simulink model "Dual_Clutch_Trans_SDO"  (R2025a)
settings: Solver=ode1  StartTime=0.0  StopTime=15  MaxStep=0.1  RelTol=1e-3  EnableMultiTasking=on
PreLoadFcn:
  | load UrbanCycle1;
  | load UrbanCycle2;
  | load UrbanCycle3;
  | load UrbanCycle4;
  | load UrbanCycle5;
  | load UrbanCycle6;
  | load UrbanCycle7;
  | load UrbanCycle8;
  | Shift_Gear_Delay = 50;
  | Ratio_Time_Const = 0.1;
  | Drive_Cycle_Num = 7;
  | load RefRPMData;
PostLoadFcn:
  | warning off Simulink:SampleTime:TsPropEnabOutputsChangeNotAligned;
  | warning off Simulink:blocks:MatchingFromNotFound
  | warning off Simulink:blocks:MatchingGotoNotFound
  | warning off Simulink:Engine:OutputNotConnected
  | warning off Simulink:Engine:LineWithoutDst
  | warning off Simulink:Engine:UINotUpdatedDuringRapidAccelSim
  | warning off Simulink:Commands:SetParamLinkChangeWarn
  | warning off Simulink:Engine:SaveWithParameterizedLinks_Warning
undefined symbols (not defined in the file or in its folder): DCT_Param, Downshift_Speeds, sigbuilder_block, Upshift_Speeds
libraries: fl_lib x5, nesl_utility x4, sdl_lib x2, simulink x2, DCT_Vehicle_Dynamics_Lib x2, Engine_Lib x1, slpidlib x1
(part 1 of 2)
Description:
  | Vehicle With Dual Clutch Transmission
  | 
  | The vehicle simulated in this demo has a five-speed automatic dual-clutch
  | transmission. The transmission controller converts the pedal deflection
  | into a demanded torque. This demanded torque is then passed to the
  | engine management. The pedal deflection and the vehicle speed are also
  | used by the transmission controller to determine when the gear shifts
  | should occur. Gear shifts are implemented via the two clutches, one clutch
  | pressure being ramped up as the other clutch pressure is ramped down.
  | Gear pre-selection is used to ensure that the correct gear is fully selected
  | before the on-going clutch is enabled. Double-click on the two blocks
  | labeled "Configure for ...." to switch between variable and fixed-step solvers.
  | 
  | 
  | Copyright 2008-2025 The MathWorks, Inc.
settings Model: ParamWorkspaceSource=ReferencedWorkspace  ExtModeTrigDuration=200  ExtModeLogAll=off  TunableVars=Downshift_Speeds,Pedal_Positions,Upshift_Speeds  TunableVarsStorageClass=Auto,Auto,Auto  TunableVarsTypeQualifier=,,  Creator=MathWorks  LastModifiedBy=smiller
settings SolverCC: MaxConsecutiveZCs=10  MaxConsecutiveMinStep=5  AlgebraicLoopSolver=TrustRegion  AutoInsertRateTranBlk=on
settings DataIOCC: LimitDataPoints=on  MaxDataPoints=1  SaveFormat=StructureWithTime  SaveOutput=off  DSMLogging=off  SaveTime=off  ReturnWorkspaceOutputs=off  SignalLoggingName=SDO_logsout
settings OptimizationCC: BlockReduction=off  OptimizeBlockIOStorage=off  BufferReuse=off  ReuseModelBlockBuffer=off  GlobalBufferReuse=off  ExpressionFolding=off  ExpressionDepthLimit=2147483647.0  LocalBlockOutputs=off  OptimizeDataStoreBuffers=off  BusAssignmentInplaceUpdate=off
settings DebuggingCC: AlgebraicLoopMsg=error  UnderspecifiedInitializationDetection=Classic  MergeDetectMultiDrivingBlocksExec=none  IgnoredZcDiagnostic=none  MultiTaskRateTransMsg=warning  FcnCallInpInsideContextMsg=warning  UnconnectedInputMsg=warning  UnconnectedOutputMsg=warning  UnconnectedLineMsg=warning  AllowSymbolicDim=off  StateNameClashWarn=warning  PregeneratedLibrarySubsystemCodeDiagnostic=none  SFUnexpectedBacktrackingDiag=warning  SFNoUnconditionalDefaultTransitionDiag=warning  SFExecutionAtInitializationDiag=none  ArithmeticOperatorsInVariantConditions=warning
settings ModelReferenceCC: EnableRefExpFcnMdlSchedulingChecks=on  PropagateSignalLabelsOutOfModel=off
settings SFSimCC: SimUseLocalCustomCode=off  CustomCodeUndefinedFunction=UseInterfaceOnly
settings RTWCC: RTWUseLocalCustomCode=off  RTWCompilerOptimization=on  GPUComputeCapability=3.5  DLArmComputeVersion=19.05
settings CodeAppCC: StateflowObjectComments=on
settings GRTTargetCC: TargetLangStandard=C89/C90 (ANSI)
settings ConfigComp: CovMetricSettings=dw  CovSaveCumulativeToWorkspaceVar=on  CovSaveSingleToWorkspaceVar=on  CovExternalEMLEnable=off  CovSFcnEnable=off
settings SimscapeCC: ExplicitSolverDiagnosticOptions=none  SimscapeNormalizeSystem=off  SimscapeNominalValues="[{\"value\":\"10\",\"unit\":\"V\"},{\"value\":\"1\",\"unit\":\"A\"},{\"value\":\"10\",\"unit\":\"N*m\"},{\"value\":\"10\",\"unit\":\"bar\"},{\"value\":\"100\",\"unit\":\"kJ/kg\"},{\"value\":\"1\",\"unit\":\"kW\"},{\"value\":\"300\",\"unit\":\"K\"},{\"value\":\"100\",\"unit\":\"cm^3/s\"},{\"value\":\"1\",\"unit\":\"kN\"},{\"value\":\"1\",\"unit\":\"g/cm^3\"},{\"value\":\"1\",\"unit\":\"l\"},{\"value\":\"1\",\"unit\":\"cm^2\"},{\"value\":\"60\",\"unit\":\"Hz\"}]"  SimscapeLogLimitData=off  SimscapeLogDataHistory=50000.0

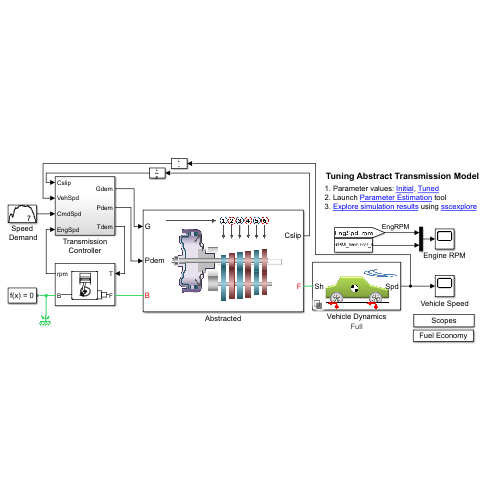
[thumbnail: Simulink's stored preview of the top-level diagram]
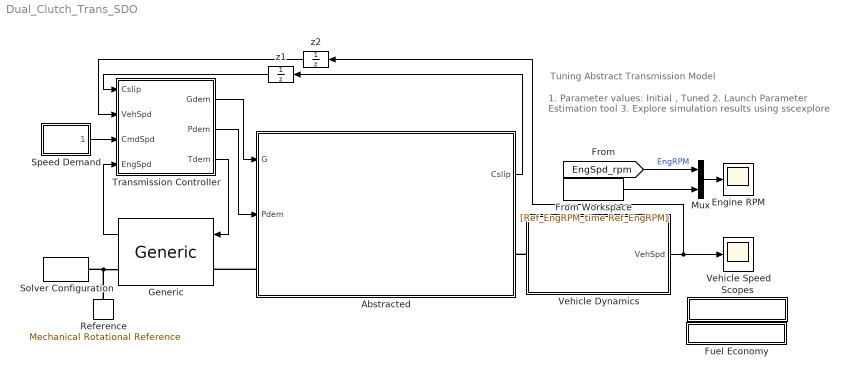
== system Dual_Clutch_Trans_SDO ==
  note: 1. Parameter values: Initial , Tuned
      | 2. Launch Parameter Estimation tool
      | 3. Explore simulation results using sscexplore
  note: Tuning Abstract Transmission Model
  Abstracted : Subsystem
      mask Display:
      | image(imread('DCT_Transmission_Abstracted_IMAGE2.jpg'));
      | port_label('input',1,'G')
      | port_label('input',2,'Pdem')
      | port_label('output',1,'Cslip')
      | color('red');
      | port_label('LConn',1,'B')
      | port_label('RConn',1,'F')
  Engine RPM : Scope
      settings: ActiveDisplayYMinimum=0  ActiveDisplayYMaximum=3000  DataLoggingMaxPoints=50000  DataLoggingVariableName=EngineRPM
  From Workspace : FromWorkspace  VariableName=[Ref_EngRPM_time Ref_EngRPM]  SampleTime=0.01
  Fuel Economy : Subsystem  mask(Data Acquisition){}
      mask Display: disp('Fuel Economy');
  Generic : Engine_Lib/Generic  SystemSampleTime=-1  VariantActivationTime=update diagram  EmptyChoice=off  PassThrough=off  PassThroughVariantControl=(default)  EmptyChoiceVariantControl=(default)  AllowFlexibleInterface=on  Latency=0  AutoFrameSizeCalculation=off
  Mux : Mux  Inputs=2
  Reference : fl_lib/Mechanical/Rotational Elements/Mechanical Rotational Reference
  Scopes : Subsystem
      mask Display: disp('Scopes')
  Solver Configuration : nesl_utility/Solver Configuration  PhysicalDomain=network_engine_domain  SubClassName=solver  LeftPortType=input  RightPortType=generic  Tones=[]  Harmonics=[]  SimulateNoise=off  Profile=off  UseLocalSampling=off  EnableSwitchedLinearOptims=on  FrequencyDomain=off  UseCCode=off  RelTol=0.001  AbsTol=1e-06  MinStep=1e-09  ToWorkspace=off  RevertToSquareIcSolve=off  NumHomotopyIterations=100  PhasorMode=off  PhasorModeNumHarmonics=1  ConsistencySolver=NEWTON_FTOL  IndexReductionMethod=DerivativeReplacement  DoDC=off  ResidualTolerance=1e-9  ConsistencyTolSource=GLOBAL  ConsistencyAbsTol=0.001  ConsistencyRelTol=0.001  ConsistencyTolFactor=0.001  UseLocalSolver=on  LocalSolverChoice=NE_BACKWARD_EULER_ADVANCER  ResolveIndetEquations=on  FunctionEvalNumThread=1  LocalSolverSampleTime=.005  DoFixedCost=on  MaxNonlinIter=2  MaxModeIter=2  ComputeImpulses=off  ImpulseIterations=2  LinearAlgebra=Sparse  LinearAlgebraNumThread=0  EquationFormulation=NE_TIME_EF  DelaysMemoryBudget=1024  AutomaticFiltering=on  FilteringTimeConstant=0.001  PartitionStorageMethod=AS_NEEDED  PartitionMemoryBudget=1024  PartitionMethod=FAST  MultibodyUseLocalSolver=off  MultibodyLocalSolverChoice=ODE1  MultibodyLocalSolverSampleTime=0.001
  Speed Demand : Subsystem
      mask Display:
      | plotstr=['UrbanCycle' evalin('base','num2str(Drive_Cycle_Num)')];
      | plot(evalin('base',[plotstr '.time']),evalin('base',[plotstr '.SpdKph']));
      | text(evalin('base',['0.7*max(' plotstr '.time)']),evalin('base',['0.25*max(' plotstr '.SpdKph)']),evalin('base','num2str(Drive_Cycle_Num)'));
  Transmission Controller : Subsystem
  Vehicle Dynamics : Subsystem  Variant=on  VariantControlMode=label  LabelModeActiveChoice=Full
      settings: AttributesFormatString=%<ActiveVariant>
      mask Display:
      | blk = Dual_Clutch_activeVariantBlock(gcb);
      | eval(get_param(blk, 'MaskDisplay'));
  Vehicle Speed : Scope
      settings: ActiveDisplayYMaximum=100  DataLoggingMaxPoints=50000  DataLoggingVariableName=VehSpd
  z1 : UnitDelay  SampleTime=0.01  HasFrameUpgradeWarning=on
  z2 : UnitDelay  SampleTime=0.01  HasFrameUpgradeWarning=on
  wires:
  Transmission Controller/2(Pdem) -> Abstracted/2(Pdem)
  Transmission Controller/1(Gdem) -> Abstracted/1(G)
  z1/1 -> Transmission Controller/1(Cslip)
  Generic/1 -> Transmission Controller/4(EngSpd)
  Abstracted/1(Cslip) -> z1/1
  Vehicle Dynamics/1(VehSpd) -> Vehicle Speed/1, z2/1
  Speed Demand/1(Speed Command) -> Transmission Controller/3(CmdSpd)
  z2/1 -> Transmission Controller/2(VehSpd)
  [EngSpd_rpm] -> Mux/1  "EngRPM"
  From Workspace/1 -> Mux/2
  Mux/1 -> Engine RPM/1
  Transmission Controller/3(Tdem) -> Generic/1
  connections:
  Generic/RConn1 -- Reference/LConn1 -- Solver Configuration/RConn1
  Abstracted/LConn1 -- Generic/LConn1
  Vehicle Dynamics/LConn1 -- Abstracted/RConn1

== system Dual_Clutch_Trans_SDO/Abstracted ==
  G : Inport
  Pdem : Inport  Port=2
  Clutches : Subsystem
      mask Display: image(imread('DCT_Clutches_Abstracted_IMAGE.jpg'));
  Gears : Subsystem
      mask Display: image(imread('DCT_Gears_Abstracted_IMAGE.jpg'));
  Shaft Inertia Output Shaft : fl_lib/Mechanical/Rotational Elements/Inertia  inertia=DCT_Param.Transmission.Shaft_Inertia_Output kg*m^2  num_ports=foundation.enum.numPorts2.one  w_specify=on  w_priority=High  w=DCT_Param.Transmission.Shaft_Velocity_Output rad/s  w_nominal_specify=off  w_nominal_value=1  w_nominal_unit=rad/s  t_specify=off  t_priority=High  t=0 N*m  t_nominal_specify=off  t_nominal_value=1  t_nominal_unit=N*m
  B : PMIOPort  Side=Left
  F : PMIOPort  Port=2  Side=Right
  Cslip : Outport  VectorParamsAs1DForOutWhenUnconnected=off
  wires:
  Pdem/1 -> Clutches/1(Pdem)
  Clutches/1(Cslip) -> Cslip/1
  G/1 -> Gears/1(G)
  connections:
  B/RConn1 -- Clutches/LConn1
  Clutches/RConn1 -- Gears/LConn1
  Gears/RConn1 -- F/RConn1 -- Shaft Inertia Output Shaft/LConn1

== system Dual_Clutch_Trans_SDO/Fuel Economy ==
  note: Fuel Economy
  (L/100 km) : Display
      settings: Decimation=decimation
  (MPG) : Display
      settings: Decimation=decimation
  (km/L) : Display
      settings: Decimation=decimation
  Calculate Fuel Economy : Subsystem
  Fuel Flow : Scope
      settings: ActiveDisplayYMinimum=0  ActiveDisplayYMaximum=7000  DataLoggingMaxPoints=50000  DataLoggingVariableName=Fuel_Flow_DATA
  Total Fuel Used (L) : Display
      settings: Decimation=decimation
  wires:
  [Fuel_Flow_gps] -> Fuel Flow/1, Calculate Fuel Economy/2(Fuel Flow g/s)
  Calculate Fuel Economy/2(Km/Liter) -> (km/L)/1
  Calculate Fuel Economy/4(Fuel Used (L)) -> Total Fuel Used (L)/1
  [VehSpd] -> Calculate Fuel Economy/1(Kph)
  Calculate Fuel Economy/3(MPG) -> (MPG)/1
  Calculate Fuel Economy/1(Liter/100Km) -> (L/100 km)/1

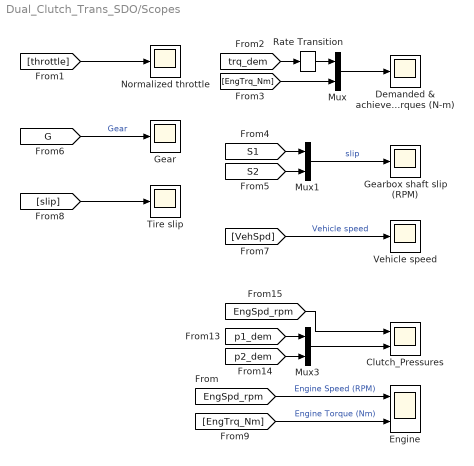
== system Dual_Clutch_Trans_SDO/Scopes ==
  Clutch_Pressures : Scope  NumInputPorts=2
      settings: ActiveDisplayYMinimum=0  ActiveDisplayYMaximum=6000  DataLoggingMaxPoints=50000  DataLoggingVariableName=Torque1
  Demanded & achieved torques (N-m) : Scope
      settings: TimeSpan=30  ActiveDisplayYMinimum=0  ActiveDisplayYMaximum=200  DataLoggingMaxPoints=50000  DataLoggingVariableName=Torque  DataLoggingSaveFormat=Array
  Engine : Scope  NumInputPorts=2
      settings: ActiveDisplayYMinimum=0  ActiveDisplayYMaximum=6000  DataLoggingMaxPoints=50000  DataLoggingVariableName=Engine_DATA
  Gear : Scope
      settings: ActiveDisplayYMinimum=0  ActiveDisplayYMaximum=5.5  DataLoggingMaxPoints=50000  DataLoggingVariableName=CurrentGear_DATA
  Gearbox shaft slip (RPM) : Scope
      settings: ActiveDisplayYMinimum=-4000  ActiveDisplayYMaximum=4000  DataLoggingMaxPoints=50000
  Mux : Mux  Inputs=2
  Mux1 : Mux  Inputs=2
  Mux3 : Mux  Inputs=2
  Normalized throttle : Scope
      settings: TimeSpan=30  ActiveDisplayYMinimum=0  ActiveDisplayYMaximum=1  DataLoggingMaxPoints=50000
  Rate Transition : RateTransition
  Tire slip : Scope
      settings: ActiveDisplayYMinimum=0  ActiveDisplayYMaximum=0.04  DataLoggingMaxPoints=500000  DataLoggingVariableName=TireSlip  DataLoggingSaveFormat=Array
  Vehicle speed : Scope
      settings: ActiveDisplayYMaximum=50  DataLoggingMaxPoints=50000  DataLoggingVariableName=VehicleSpeed_DATA
  wires:
  [throttle] -> Normalized throttle/1
  Mux/1 -> Demanded & achieved torques (N-m)/1
  [EngTrq_Nm] -> Mux/2
  Mux1/1 -> Gearbox shaft slip (RPM)/1  "slip"
  [S1] -> Mux1/1
  [S2] -> Mux1/2
  [G] -> Gear/1  "Gear"
  [VehSpd] -> Vehicle speed/1  "Vehicle speed"
  [slip] -> Tire slip/1
  Mux3/1 -> Clutch_Pressures/2
  [p1_dem] -> Mux3/1
  [p2_dem] -> Mux3/2
  [EngSpd_rpm] -> Clutch_Pressures/1
  [trq_dem] -> Rate Transition/1
  Rate Transition/1 -> Mux/1
  [EngSpd_rpm] -> Engine/1  "Engine Speed (RPM)"
  [EngTrq_Nm] -> Engine/2  "Engine Torque (Nm)"

== system Dual_Clutch_Trans_SDO/Speed Demand ==
  "10-15 mode " : Subsystem  Tag=STV Subsys  LoadFcn=sigbuilder_block('load');  StartFcn=sigbuilder_block('start');  StopFcn=sigbuilder_block('stop');  ClipboardFcn=sigbuilder_block('clipboard');  mask(Sigbuilder block){tuvar=[0:10]}
      mask help: Sigbuilder GUI
      mask init:
      | if ~strcmp(get_param(bdroot(gcbh),'SimulationStatus'),'stopped') tuvar = sigbuilder_block('maskInit'); end
      settings: CopyFcn=sigbuilder_block('copy');  DeleteFcn=sigbuilder_block('delete');  ModelCloseFcn=sigbuilder_block('modelClose');  PreSaveFcn=sigbuilder_block('preSave');  PauseFcn=sigbuilder_block('pause')  ContinueFcn=sigbuilder_block('continue')  NameChangeFcn=sigbuilder_block('namechange');  OpenFcn=sigbuilder_block('open',[561.75 178.5 550.5 399 ]);  CloseFcn=sigbuilder_block('close');
      mask Display: plot(0, 0, 100, 100,[2, 2, 32, 32, 2], [68, 8, 8, 68, 68],[32, 2], [38, 38], [32, 19, 2],[53, 60, 44], [32, 17, 17, 2],[16, 16, 31, 31]);txt = getActiveGroup(gcbh);text(2, 100, txt,'verticalAlignment', 'top');
  FTP75 : FromWorkspace  VariableName=[UrbanCycle4.time UrbanCycle4.SpdKph]
  FTP75 Transient : FromWorkspace  VariableName=[UrbanCycle8.time UrbanCycle8.SpdKph]
  FTP75 short : FromWorkspace  VariableName=[UrbanCycle7.time UrbanCycle7.SpdKph]
  Multiport Switch : MultiPortSwitch  Inputs=8  SaturateOnIntegerOverflow=off  InputSameDT=off
  Select Cycle : Constant  Value=Drive_Cycle_Num
  Urban Cycle 1 : FromWorkspace  VariableName=[UrbanCycle1.time UrbanCycle1.SpdKph]
  Urban Cycle 2 : FromWorkspace  VariableName=[UrbanCycle2.time UrbanCycle2.SpdKph]
  Urban Cycle 3 : FromWorkspace  VariableName=[UrbanCycle3.time UrbanCycle3.SpdKph]
  Wide Open Throttle : FromWorkspace  VariableName=[UrbanCycle4.time UrbanCycle4.SpdKph]
  Speed Command : Outport  VectorParamsAs1DForOutWhenUnconnected=off
  wires:
  Urban Cycle 3/1 -> Multiport Switch/4
  Select Cycle/1 -> Multiport Switch/1
  Urban Cycle 2/1 -> Multiport Switch/3
  Urban Cycle 1/1 -> Multiport Switch/2
  FTP75/1 -> Multiport Switch/5
  "10-15 mode "/1(Target speed) -> Multiport Switch/6
  Multiport Switch/1 -> Speed Command/1
  FTP75 short/1 -> Multiport Switch/8
  Wide Open Throttle/1 -> Multiport Switch/7
  FTP75 Transient/1 -> Multiport Switch/9

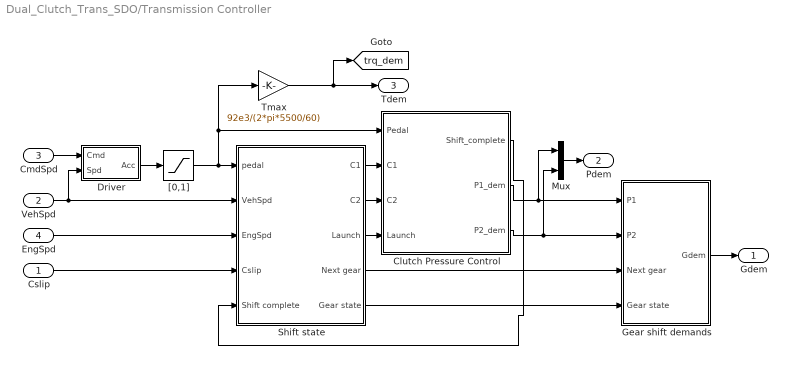
== system Dual_Clutch_Trans_SDO/Transmission Controller ==
  Cslip : Inport
  VehSpd : Inport  Port=2
  CmdSpd : Inport  Port=3
  EngSpd : Inport  Port=4
  Clutch Pressure Control : Subsystem
  Driver : Subsystem
  Gear shift demands : Subsystem
  Mux : Mux  Inputs=2
  Shift state : Subsystem
  Tmax : Gain  Gain=92e3/(2*pi*5500/60)  SaturateOnIntegerOverflow=on  OutDataTypeStr=Inherit: Same as input  ParamDataTypeStr=Inherit: Same as input
  "[0,1]" : Saturate  UpperLimit=1  LowerLimit=0
  Gdem : Outport  VectorParamsAs1DForOutWhenUnconnected=off
  Pdem : Outport  Port=2  VectorParamsAs1DForOutWhenUnconnected=off
  Tdem : Outport  Port=3  VectorParamsAs1DForOutWhenUnconnected=off
  tag scope: trq_dem=global
  wires:
  "[0,1]"/1 -> Shift state/1(pedal), Clutch Pressure Control/1(Pedal), Tmax/1
  VehSpd/1 -> Shift state/2(VehSpd), Driver/2(Spd)
  EngSpd/1 -> Shift state/3(EngSpd)
  Cslip/1 -> Shift state/4(Cslip)
  Shift state/5(Gear state) -> Gear shift demands/4(Gear state)
  Shift state/4(Next gear) -> Gear shift demands/3(Next gear)
  Gear shift demands/1(Gdem) -> Gdem/1
  Shift state/1(C1) -> Clutch Pressure Control/2(C1)
  Shift state/2(C2) -> Clutch Pressure Control/3(C2)
  Shift state/3(Launch) -> Clutch Pressure Control/4(Launch)
  Clutch Pressure Control/1(Shift_complete) -> Shift state/5(Shift complete)
  Clutch Pressure Control/3(P2_dem) -> Gear shift demands/2(P2), Mux/2
  Clutch Pressure Control/2(P1_dem) -> Gear shift demands/1(P1), Mux/1
  Tmax/1 -> Tdem/1, [trq_dem]
  Mux/1 -> Pdem/1
  CmdSpd/1 -> Driver/1(Cmd)
  Driver/1(Acc) -> "[0,1]"/1

== system Dual_Clutch_Trans_SDO/Vehicle Dynamics ==
  note: Variant Subsystems
  Full : DCT_Vehicle_Dynamics_Lib/Full  SystemSampleTime=-1  VariantControl=Full  VariantActivationTime=update diagram  EmptyChoice=off  PassThrough=off  PassThroughVariantControl=(default)  EmptyChoiceVariantControl=(default)  AllowFlexibleInterface=on  Latency=0  AutoFrameSizeCalculation=off
  Simple : DCT_Vehicle_Dynamics_Lib/Simple  VariantControl=Simple  mass=DCT_Param.Vehicle.Mass  area=DCT_Param.Vehicle.Frontal_Area  Cd=DCT_Param.Vehicle.Aero_Drag_Coeff  radius=DCT_Param.Vehicle.Tire.Radius  wheel_inertia=DCT_Param.Vehicle.Tire.Inertia  gear_ratio=DCT_Param.Vehicle.Final_Drive_Ratio
  Drive Shaft : PMIOPort  Side=Left
  VehSpd : Outport  VectorParamsAs1DForOutWhenUnconnected=off

== system Dual_Clutch_Trans_SDO/Abstracted/Clutches ==
  Pdem : Inport
  Clutch Odd Gears : sdl_lib/Clutches/Disc Friction Clutch  geometry_model=1  r_eff=DCT_Param.Clutch.Torque_Radius mm  d_o=150 mm  d_i=100 mm  nS=DCT_Param.Clutch.Num_Friction_Surfaces  piston_area=DCT_Param.Clutch.Engagement_Piston_Area m^2  unidirectional=0  friction_model=1  mu_w_vector=[ 0 0.1 0.2 0.3 0.4 0.5 1 2 5 10 100 1000 ] rad/s  temperature_TLU=[280.0, 300.0, 320.0] K  mu_static=DCT_Param.Clutch.Static_Friction_Coeff  mu_static_vector=[0.4, 0.38, 0.36]  mu_coulomb=DCT_Param.Clutch.Kinetic_Friction_Coeff  mu_coulomb_vector=[ 0.29 0.28 0.26 0.22 0.21 0.2 0.2 0.19 0.19 0.19 0.19 0.19 ]  mu_coulomb_temp_vector=[0.3, 0.28, 0.25]  mu_coulomb_matrix=[0.34, 0.32, 0.3; 0.3, 0.28, 0.25; 0.25, 0.2, 0.15]  mu_interp_method=1  mu_extrap_method=1  d_f=DCT_Param.Clutch.Derating_Factor  w_tol=DCT_Param.Clutch.Clutch_Velocity_Tolerance rad/s  pressure_min=DCT_Param.Clutch.Threshold_Pressure Pa  mu_visc=DCT_Param.Clutch.Drag_Torque_Coeff N*m/(rad/s)  initial_state_locked=0  thermal_mass=25 kJ/K  T_init=300 K
      settings: InternalSimscapePortConfiguration="{\"Bottom\":[],\"Left\":[{\"id\":\"P\",\"label\":\"P\",\"type\":\"input\"},{\"id\":\"B\",\"label\":\"B\",\"type\":\"foundation.mechanical.rotational.rotational\"}],\"Right\":[{\"id\":\"F\",\"label\":\"F\",\"type\":\"foundation.mechanical.rotational.rotational\"}],\"Top\":[]}"
  MinMax : MinMax  Function=max
  Mux : Mux  Inputs=2
  Odd Clutch Actuator : Subsystem
  Shaft Inertia All Gears : fl_lib/Mechanical/Rotational Elements/Inertia  inertia=DCT_Param.Transmission.Shaft_Inertia_Odd kg*m^2  num_ports=foundation.enum.numPorts2.one  w_specify=on  w_priority=High  w=DCT_Param.Transmission.Shaft_Velocity_Odd rad/s  w_nominal_specify=off  w_nominal_value=1  w_nominal_unit=rad/s  t_specify=off  t_priority=High  t=0 N*m  t_nominal_specify=off  t_nominal_value=1  t_nominal_unit=N*m
  Slip Sensor 2 : Constant  Value=0
  Slip sensor 1 : Subsystem
  Shaft : PMIOPort  Side=Right
  E : PMIOPort  Port=2  Side=Left
  Cslip : Outport  VectorParamsAs1DForOutWhenUnconnected=off
  wires:
  Slip sensor 1/1(S1) -> Mux/1
  Mux/1 -> Cslip/1
  Pdem/1 -> MinMax/1
  MinMax/1 -> Odd Clutch Actuator/1(Pdem)
  Slip Sensor 2/1 -> Mux/2
  connections:
  E/RConn1 -- Slip sensor 1/LConn1 -- Clutch Odd Gears/LConn2
  Odd Clutch Actuator/RConn1 -- Clutch Odd Gears/LConn1
  Slip sensor 1/RConn1 -- Clutch Odd Gears/RConn1 -- Shaft/RConn1 -- Shaft Inertia All Gears/LConn1

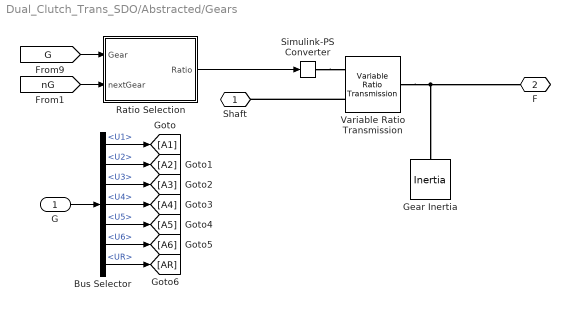
== system Dual_Clutch_Trans_SDO/Abstracted/Gears ==
  G : Inport
  Bus Selector : BusSelector  OutputSignals=U1,U2,U3,U4,U5,U6,UR
  Gear Inertia : fl_lib/Mechanical/Rotational Elements/Inertia  inertia=DCT_Param.Transmission.Gear_Inertia kg*m^2  num_ports=foundation.enum.numPorts2.one  w_specify=on  w_priority=High  w=0 rad/s  w_nominal_specify=off  w_nominal_value=1  w_nominal_unit=rad/s  t_specify=off  t_priority=High  t=0 N*m  t_nominal_specify=off  t_nominal_value=1  t_nominal_unit=N*m
  Ratio Selection : Subsystem
  Simulink-PS Converter : nesl_utility/Simulink-PS Converter  PhysicalDomain=network_engine_domain  SubClassName=ps_input  LeftPortType=input  RightPortType=output  PseudoPeriodic=off  Frequencies=[]  NoiseDistribution=none  NoiseParameters=[]  Unit=1  AffineConversion=off  FilteringAndDerivatives=zero  SimscapeFilterOrder=1  InputFilterTimeConstant=0.005  UdotUserProvided=0
  Variable Ratio Transmission : sdl_lib/Couplings & Drives/Variable Ratio Transmission  rotation_direction=3-2*(2)  kp=DCT_Param.Transmission.Abstract.Compliance N*m/rad  kv=DCT_Param.Transmission.Abstract.Damping N*m/(rad/s)  initial_torque=0 N*m  ratio_thr=0.01  losses_model=(1)-1  efficiency=0.85  pwr_thr=0.001 W  mu_visc=[ 0 0 ] N*m/(rad/s)
      settings: InternalSimscapePortConfiguration="{\"Bottom\":[],\"Left\":[{\"id\":\"ratio\",\"label\":\"r\",\"type\":\"input\"},{\"id\":\"B\",\"label\":\"B\",\"type\":\"foundation.mechanical.rotational.rotational\"}],\"Right\":[{\"id\":\"F\",\"label\":\"F\",\"type\":\"foundation.mechanical.rotational.rotational\"}],\"Top\":[]}"
  Shaft : PMIOPort  Side=Left
  F : PMIOPort  Port=2  Side=Right
  wires:
  [nG] -> Ratio Selection/2(nextGear)
  G/1 -> Bus Selector/1
  Bus Selector/1 -> [A1]  "<U1>"
  Bus Selector/2 -> [A2]  "<U2>"
  Bus Selector/3 -> [A3]  "<U3>"
  Bus Selector/4 -> [A4]  "<U4>"
  Bus Selector/5 -> [A5]  "<U5>"
  Bus Selector/6 -> [A6]  "<U6>"
  Bus Selector/7 -> [AR]  "<UR>"
  Ratio Selection/1(Ratio) -> Simulink-PS Converter/1
  [G] -> Ratio Selection/1(Gear)
  connections:
  Variable Ratio Transmission/LConn2 -- Shaft/RConn1
  Variable Ratio Transmission/RConn1 -- Gear Inertia/LConn1 -- F/RConn1
  Simulink-PS Converter/RConn1 -- Variable Ratio Transmission/LConn1

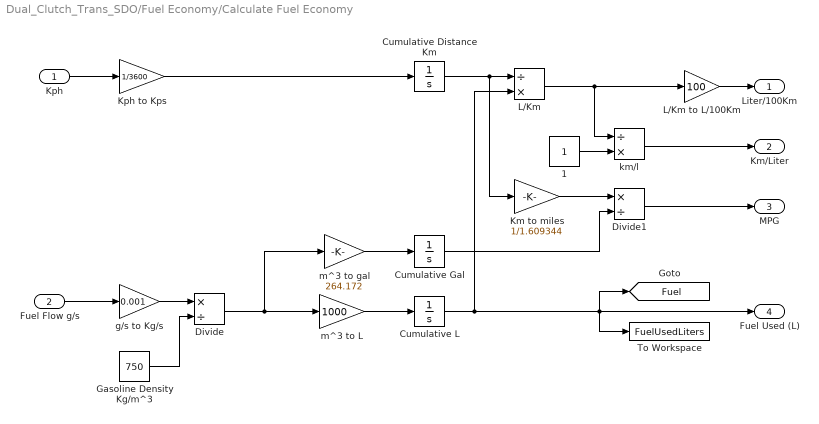
== system Dual_Clutch_Trans_SDO/Fuel Economy/Calculate Fuel Economy ==
  Kph : Inport
  Fuel Flow g/s : Inport  Port=2
  1 : Constant
  Cumulative Distance Km : Integrator  InitialCondition=eps
  Cumulative Gal : Integrator  InitialCondition=eps
  Cumulative L : Integrator  InitialCondition=eps
  Divide : Product  Inputs=*/
  Divide1 : Product  Inputs=*/
  Gasoline Density Kg/m^3 : Constant  Value=750
  Km to miles : Gain  Gain=1/1.609344
  Kph to Kps : Gain  Gain=1/3600
  L/Km : Product  Inputs=/*
  L/Km to L/100Km : Gain  Gain=100
  To Workspace : ToWorkspace  VariableName=FuelUsedLiters  SampleTime=-1
      settings: MaxDataPoints=1
  g/s to Kg/s : Gain  Gain=0.001
  km/l : Product  Inputs=/*
  m^3 to L : Gain  Gain=1000
  m^3 to gal : Gain  Gain=264.172
  Liter/100Km : Outport  VectorParamsAs1DForOutWhenUnconnected=off
  Km/Liter : Outport  Port=2  VectorParamsAs1DForOutWhenUnconnected=off
  MPG : Outport  Port=3  VectorParamsAs1DForOutWhenUnconnected=off
  Fuel Used (L) : Outport  Port=4  VectorParamsAs1DForOutWhenUnconnected=off
  tag scope: Fuel=global
  wires:
  g/s to Kg/s/1 -> Divide/1
  Gasoline Density Kg/m^3/1 -> Divide/2
  Divide/1 -> m^3 to L/1, m^3 to gal/1
  m^3 to L/1 -> Cumulative L/1
  m^3 to gal/1 -> Cumulative Gal/1
  Kph to Kps/1 -> Cumulative Distance Km/1
  Cumulative L/1 -> [Fuel], To Workspace/1, Fuel Used (L)/1, L/Km/2
  Cumulative Distance Km/1 -> L/Km/1, Km to miles/1
  L/Km/1 -> L/Km to L/100Km/1, km/l/1
  Km to miles/1 -> Divide1/1
  Cumulative Gal/1 -> Divide1/2
  Kph/1 -> Kph to Kps/1
  Fuel Flow g/s/1 -> g/s to Kg/s/1
  L/Km to L/100Km/1 -> Liter/100Km/1
  Divide1/1 -> MPG/1
  1/1 -> km/l/2
  km/l/1 -> Km/Liter/1

== system Dual_Clutch_Trans_SDO/Speed Demand/10-15 mode  ==
  Demux : Demux  Tag=STV Demux  Outputs=1
      settings: DisplayOption=none
  FromWs : FromWorkspace  Tag=STV FromWs  VariableName=tuvar
      SigBuilderData=|
      | common.afterFinalStr = 'Extrapolate'
      | common.sampleTime = '0'
      | dataSet.timeRange = [0 660]
      | dataSet.name = '10-15 Mode Cycle'
      | sbobj.Groups.Name = '10-15 Mode Cycle'
      | sbobj.Groups.Signals.Name = 'Target speed'
      | sbobj.Groups.Signals.XData = [0 44 51 66 73 89 103 118 128 130 142 152 159 179 186 201 208 224 238 253 263 265 277 287 294 314 321 336 343 359 373 388 398 400 412 422 429 494 512 524 528 532 548 558 569 579 589 593 615 620 640 650 660]
      | sbobj.Groups.Signals.YData = [0 0 20 20 0 0 40 40 20 20 40 20 0 0 20 20 0 0 40 40 20 20 40 20 0 0 20 20 0 0 40 40 20 20 40 20 0 0 50 50 40 40 60 60 70 70 50 50 70 70 30 0 0]
  Target speed : Outport  Tag=STV Outport  VectorParamsAs1DForOutWhenUnconnected=off
  wires:
  Demux/1 -> Target speed/1
  FromWs/1 -> Demux/1

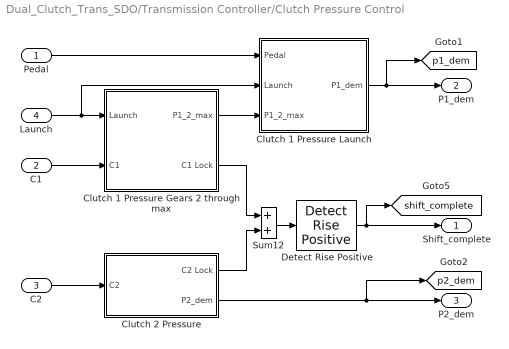
== system Dual_Clutch_Trans_SDO/Transmission Controller/Clutch Pressure Control ==
  Pedal : Inport
  C1 : Inport  Port=2
  C2 : Inport  Port=3
  Launch : Inport  Port=4
  Clutch 1 Pressure Gears 2 through max : Subsystem
  Clutch 1 Pressure Launch : Subsystem
  Clutch 2 Pressure : Subsystem
  Detect Rise Positive : simulink/Logic and Bit Operations/Detect Rise Positive  vinit=0  OutDataTypeStr=uint8
  Sum12 : Sum  InputSameDT=on  SaturateOnIntegerOverflow=on  OutDataTypeStr=Inherit: Same as first input
  Shift_complete : Outport  OutputWhenDisabled=reset  InitialOutput=0  VectorParamsAs1DForOutWhenUnconnected=off
  P1_dem : Outport  Port=2  OutputWhenDisabled=reset  InitialOutput=0  VectorParamsAs1DForOutWhenUnconnected=off
  P2_dem : Outport  Port=3  OutputWhenDisabled=reset  InitialOutput=0  VectorParamsAs1DForOutWhenUnconnected=off
  tag scope: p1_dem=global, p2_dem=global, shift_complete=global
  wires:
  C2/1 -> Clutch 2 Pressure/1(C2)
  Clutch 2 Pressure/2(P2_dem) -> [p2_dem], P2_dem/1
  Clutch 1 Pressure Launch/1(P1_dem) -> P1_dem/1, [p1_dem]
  Sum12/1 -> Detect Rise Positive/1
  Detect Rise Positive/1 -> Shift_complete/1, [shift_complete]
  Clutch 1 Pressure Gears 2 through max/1(P1_2_max) -> Clutch 1 Pressure Launch/3(P1_2_max)
  C1/1 -> Clutch 1 Pressure Gears 2 through max/2(C1)
  Launch/1 -> Clutch 1 Pressure Gears 2 through max/1(Launch), Clutch 1 Pressure Launch/2(Launch)
  Clutch 1 Pressure Gears 2 through max/2(C1 Lock) -> Sum12/1
  Pedal/1 -> Clutch 1 Pressure Launch/1(Pedal)
  Clutch 2 Pressure/1(C2 Lock) -> Sum12/2

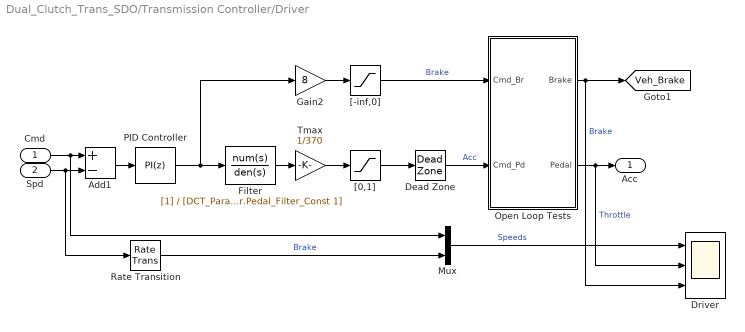
== system Dual_Clutch_Trans_SDO/Transmission Controller/Driver ==
  Cmd : Inport
  Spd : Inport  Port=2
  Add1 : Sum  Inputs=+-  SampleTime=0.01
  Dead Zone : DeadZone  LowerValue=0  UpperValue=2e-2
  Driver : Scope  NumInputPorts=3
      settings: ActiveDisplayYMinimum=-5  ActiveDisplayYMaximum=35  DataLoggingMaxPoints=50000  DataLoggingVariableName=Driver_DATA
  Filter : TransferFcn  Denominator=[DCT_Param.Driver.Pedal_Filter_Const 1]
  Gain2 : Gain  Gain=8
  Mux : Mux  Inputs=2
  Open Loop Tests : Subsystem
  PID Controller : slpidlib/PID Controller  Controller=PI  Form=Parallel  TimeDomain=Discrete-time  UseExternalTs=off  SampleTime=-1  IntegratorMethod=Forward Euler  FilterMethod=Forward Euler  ControllerParametersSource=internal  P=DCT_Param.Driver.Kp  I=DCT_Param.Driver.Ki  UseKiTs=off  D=0  UseExternalDerivativeSource=off  N=100  UseFilter=on  TunerSelectOption=Transfer Function Based (PID Tuner App)  InitialConditionSource=internal  InitialConditionForIntegrator=0  InitialConditionForFilter=0  DifferentiatorICPrevScaledInput=0  ExternalReset=none  TrackingMode=off  Kt=1  LimitOutput=off  SatLimitsSource=internal  UpperSaturationLimit=inf  LowerSaturationLimit=-inf  LinearizeAsGain=off  AntiWindupMode=none  Kb=1  LimitIntegrator=off  UpperIntegratorSaturationLimit=inf  LowerIntegratorSaturationLimit=-inf  POutMin=[]  POutMax=[]  IOutMin=[]  IOutMax=[]  DOutMin=[]  DOutMax=[]  NOutMin=[]  NOutMax=[]  SumOutMin=[]  SumOutMax=[]  SaturationOutMin=[]  SaturationOutMax=[]  PParamMin=[]  PParamMax=[]  IParamMin=[]  IParamMax=[]  DParamMin=[]  DParamMax=[]  NParamMin=[]  NParamMax=[]  KbParamMin=[]  KbParamMax=[]  KtParamMin=[]  KtParamMax=[]  KbOutMin=[]  KbOutMax=[]  KtOutMin=[]  KtOutMax=[]  IntegratorOutMin=[]  IntegratorOutMax=[]  FilterOutMin=[]  FilterOutMax=[]  SumI1OutMin=[]  SumI1OutMax=[]  SumI2OutMin=[]  SumI2OutMax=[]  SumI3OutMin=[]  SumI3OutMax=[]  SumI4OutMin=[]  SumI4OutMax=[]  SumDOutMin=[]  SumDOutMax=[]  DifferentiatorOutMin=[]  DifferentiatorOutMax=[]  FilterDiffOutCoefMin=[]  FilterDiffOutCoefMax=[]  ReciprocalOutMin=[]  ReciprocalOutMax=[]  SumDenOutMin=[]  SumDenOutMax=[]  SumNumOutMin=[]  SumNumOutMax=[]  DivideOutMin=[]  DivideOutMax=[]  UdiffTsProdOutMin=[]  UdiffTsProdOutMax=[]  NTsProdOutMin=[]  NTsProdOutMax=[]  UintegralTsProdOutMin=[]  UintegralTsProdOutMax=[]  UngainTsProdOutMin=[]  UngainTsProdOutMax=[]  ClampingZeroOutDataTypeStr=Inherit: Inherit via back propagation  ClampingZeroOutMin=[]  ClampingZeroOutMax=[]  FilterDenConstantOutDataTypeStr=Inherit: Inherit via back propagation  FilterDenConstantOutMin=[]  FilterDenConstantOutMax=[]  PCopyOutDataTypeStr=Inherit: Inherit via back propagation  PCopyOutMin=[]  PCopyOutMax=[]  NCopyOutDataTypeStr=Inherit: Inherit via back propagation  NCopyOutMin=[]  NCopyOutMax=[]  IntegratorContinuousStateAttributes=''  IntegratorStateMustResolveToSignalObject=off  IntegratorRTWStateStorageClass=Auto  FilterContinuousStateAttributes=''  FilterStateMustResolveToSignalObject=off  FilterRTWStateStorageClass=Auto  ParallelPVariant=InternalParameters  IdealPVariant=Disabled  IVariant=InternalParameters  DVariant=Disabled  IntegratorVariant=Discrete  SatVariant=Disabled  AWVariant=Passthrough  PCopyVariant=Disabled  TRVariant=Disabled  FdbkBlocksVariant=Forward  IdealPFdbkVariant=Disabled  SatFdbkVariant=Disabled  DerivativeFilterVariant=Disabled  NVariant=Disabled  NCopyVariant=Disabled_SignalSpec  FilterICVariant=Disabled  IntegratorICVariant=InternalICs  ExternalResetVariant=Disabled  TRSumVariant=Passthrough  SumFdbkVariant=Disabled  SumVariant=Sum_PI  TsampFilterVariant=InternalTs  TsampNgainVariant=Passthrough  TsampIntegralVariant=Disabled_SignalSpec  ExternalSaturationOutDataTypeStr=Inherit: Same as second input  DerivativeSourceVariant=Disabled  PreIntVariant=InternalPreInt
  Rate Transition : RateTransition
  Tmax : Gain  Gain=1/370  SaturateOnIntegerOverflow=on  OutDataTypeStr=Inherit: Same as input  ParamDataTypeStr=Inherit: Same as input
  "[-inf,0]" : Saturate  UpperLimit=0  LowerLimit=-inf
  "[0,1]" : Saturate  UpperLimit=1  LowerLimit=0
  Acc : Outport  VectorParamsAs1DForOutWhenUnconnected=off
  tag scope: Veh_Brake=global
  wires:
  "[0,1]"/1 -> Dead Zone/1
  Cmd/1 -> Mux/1, Add1/1
  Spd/1 -> Add1/2, Rate Transition/1
  "[-inf,0]"/1 -> Open Loop Tests/1(Cmd_Br)  "Brake"
  Add1/1 -> PID Controller/1
  Tmax/1 -> "[0,1]"/1
  PID Controller/1 -> Filter/1, Gain2/1
  Open Loop Tests/1(Brake) -> Driver/3, [Veh_Brake]  "Brake"
  Mux/1 -> Driver/1  "Speeds"
  Gain2/1 -> "[-inf,0]"/1
  Dead Zone/1 -> Open Loop Tests/2(Cmd_Pd)  "Acc"
  Open Loop Tests/2(Pedal) -> Driver/2, Acc/1  "Throttle"
  Rate Transition/1 -> Mux/2  "Brake"
  Filter/1 -> Tmax/1

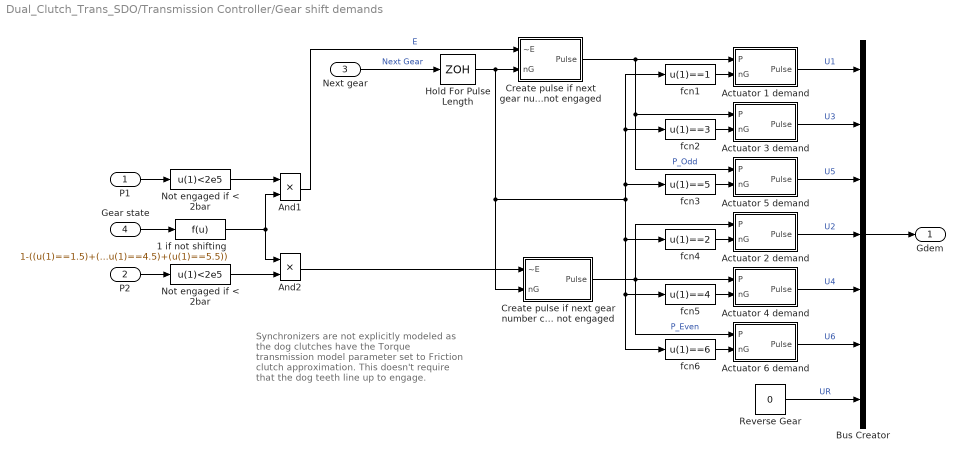
== system Dual_Clutch_Trans_SDO/Transmission Controller/Gear shift demands ==
  note: Synchronizers are not explicitly
      | modeled as the dog clutches have
      | the Torque transmission model
      | parameter set to Friction clutch
      | approximation. This doesn't require
      | that the dog teeth line up to
      | engage.
  P1 : Inport
  P2 : Inport  Port=2
  Next gear : Inport  Port=3
  Gear state : Inport  Port=4
  1 if not shifting : Fcn  Expr=1-((u(1)==1.5)+(u(1)==2.5)+(u(1)==3.5)+(u(1)==4.5)+(u(1)==5.5))
  Actuator 1 demand : Subsystem
  Actuator 2 demand : Subsystem
  Actuator 3 demand : Subsystem
  Actuator 4 demand : Subsystem
  Actuator 5 demand : Subsystem
  Actuator 6 demand : Subsystem
  And1 : Product  InputSameDT=on  SaturateOnIntegerOverflow=on  OutDataTypeStr=Inherit: Same as first input
  And2 : Product  InputSameDT=on  SaturateOnIntegerOverflow=on  OutDataTypeStr=Inherit: Same as first input
  Bus Creator : BusCreator  Inputs=7
  Create pulse if next gear number changes and CL1 is not engaged : Subsystem
  Create pulse if next gear number changes and CL2 is not engaged : Subsystem
  Hold For Pulse Length : ZeroOrderHold  SampleTime=DCT_Param.Dog_Clutches.Pulse_Length*0.01
  Not engaged if < 2bar : Fcn  Expr=u(1)<2e5
  "Not engaged if < 2bar " : Fcn  Expr=u(1)<2e5
  Reverse Gear : Constant  Value=0  SampleTime=0.01
  fcn1 : Fcn  Expr=u(1)==1
  fcn2 : Fcn  Expr=u(1)==3
  fcn3 : Fcn  Expr=u(1)==5
  fcn4 : Fcn  Expr=u(1)==2
  fcn5 : Fcn  Expr=u(1)==4
  fcn6 : Fcn  Expr=u(1)==6
  Gdem : Outport  VectorParamsAs1DForOutWhenUnconnected=off
  wires:
  And2/1 -> Create pulse if next gear number changes and CL2 is not engaged/1(~E)
  And1/1 -> Create pulse if next gear number changes and CL1 is not engaged/1(~E)  "E"
  "Not engaged if < 2bar "/1 -> And2/2
  1 if not shifting/1 -> And2/1, And1/2
  Not engaged if < 2bar/1 -> And1/1
  P2/1 -> "Not engaged if < 2bar "/1
  P1/1 -> Not engaged if < 2bar/1
  Gear state/1 -> 1 if not shifting/1
  Actuator 4 demand/1(Pulse) -> Bus Creator/5  "U4"
  Actuator 2 demand/1(Pulse) -> Bus Creator/4  "U2"
  Create pulse if next gear number changes and CL2 is not engaged/1(Pulse) -> Actuator 4 demand/1(P), Actuator 2 demand/1(P), Actuator 6 demand/1(P)  "P_Even"
  fcn5/1 -> Actuator 4 demand/2(nG)
  fcn4/1 -> Actuator 2 demand/2(nG)
  Actuator 5 demand/1(Pulse) -> Bus Creator/3  "U5"
  Actuator 3 demand/1(Pulse) -> Bus Creator/2  "U3"
  Create pulse if next gear number changes and CL1 is not engaged/1(Pulse) -> Actuator 5 demand/1(P), Actuator 3 demand/1(P), Actuator 1 demand/1(P)  "P_Odd"
  fcn3/1 -> Actuator 5 demand/2(nG)
  fcn2/1 -> Actuator 3 demand/2(nG)
  fcn1/1 -> Actuator 1 demand/2(nG)
  Next gear/1 -> Hold For Pulse Length/1  "Next Gear"
  Actuator 1 demand/1(Pulse) -> Bus Creator/1  "U1"
  Bus Creator/1 -> Gdem/1
  fcn6/1 -> Actuator 6 demand/2(nG)
  Actuator 6 demand/1(Pulse) -> Bus Creator/6  "U6"
  Reverse Gear/1 -> Bus Creator/7  "UR"
  Hold For Pulse Length/1 -> Create pulse if next gear number changes and CL1 is not engaged/2(nG), Create pulse if next gear number changes and CL2 is not engaged/2(nG), fcn4/1, fcn5/1, fcn6/1, fcn3/1, fcn2/1, fcn1/1

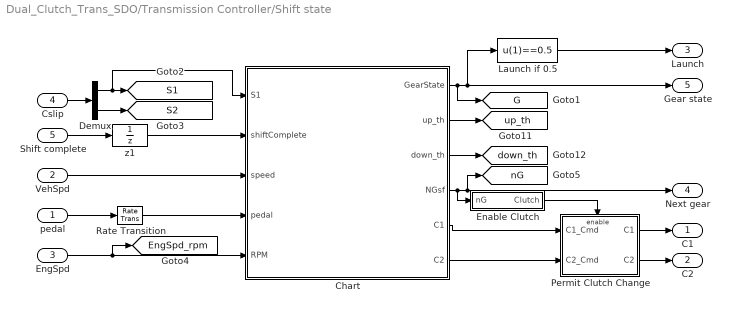
== system Dual_Clutch_Trans_SDO/Transmission Controller/Shift state ==
  pedal : Inport
  VehSpd : Inport  Port=2
  EngSpd : Inport  Port=3
  Cslip : Inport  Port=4
  Shift complete : Inport  Port=5
  Chart : Stateflow chart  TreatAsAtomicUnit=on
  Demux : Demux  Outputs=2
  Enable Clutch : Subsystem
  Launch if 0.5 : Fcn  Expr=u(1)==0.5
  Permit Clutch Change : Subsystem  TreatAsAtomicUnit=on
  Rate Transition : RateTransition  OutPortSampleTime=0.01
  z1 : UnitDelay  SampleTime=0.01  HasFrameUpgradeWarning=on
  C1 : Outport  VectorParamsAs1DForOutWhenUnconnected=off
  C2 : Outport  Port=2  VectorParamsAs1DForOutWhenUnconnected=off
  Launch : Outport  Port=3  VectorParamsAs1DForOutWhenUnconnected=off
  Next gear : Outport  Port=4  VectorParamsAs1DForOutWhenUnconnected=off
  Gear state : Outport  Port=5  VectorParamsAs1DForOutWhenUnconnected=off
  tag scope: EngSpd_rpm=global, G=global, S1=global, S2=global, down_th=global, nG=global, up_th=global
  wires:
  VehSpd/1 -> Chart/3(speed)
  EngSpd/1 -> [EngSpd_rpm], Chart/5(RPM)
  pedal/1 -> Rate Transition/1
  Shift complete/1 -> z1/1
  z1/1 -> Chart/2(shiftComplete)
  Chart/2(up_th) -> [up_th]
  Chart/3(down_th) -> [down_th]
  Chart/4(NGsf) -> [nG], Next gear/1, Enable Clutch/1(nG)
  Chart/5(C1) -> Permit Clutch Change/1(C1_Cmd)
  Chart/6(C2) -> Permit Clutch Change/2(C2_Cmd)
  Launch if 0.5/1 -> Launch/1
  Demux/1 -> [S1], Chart/1(S1)
  Demux/2 -> [S2]
  Cslip/1 -> Demux/1
  Chart/1(GearState) -> [G], Gear state/1, Launch if 0.5/1
  Enable Clutch/1(Clutch) -> Permit Clutch Change/Enable
  Permit Clutch Change/1(C1) -> C1/1
  Permit Clutch Change/2(C2) -> C2/1
  Rate Transition/1 -> Chart/4(pedal)

== system Dual_Clutch_Trans_SDO/Abstracted/Clutches/Odd Clutch Actuator ==
  Pdem : Inport
  Pressure controller time constant : TransferFcn  Denominator=[0.02 1]
  Simulink-PS Converter : nesl_utility/Simulink-PS Converter  PhysicalDomain=network_engine_domain  SubClassName=ps_input  LeftPortType=input  RightPortType=output  PseudoPeriodic=off  Frequencies=[]  NoiseDistribution=none  NoiseParameters=[]  Unit=Pa  AffineConversion=off  FilteringAndDerivatives=zero  SimscapeFilterOrder=1  InputFilterTimeConstant=0.005  UdotUserProvided=0
  P : PMIOPort  Side=Right
  wires:
  Pressure controller time constant/1 -> Simulink-PS Converter/1
  Pdem/1 -> Pressure controller time constant/1
  connections:
  P/RConn1 -- Simulink-PS Converter/RConn1

== system Dual_Clutch_Trans_SDO/Abstracted/Clutches/Slip sensor 1 ==
  Ideal Rotational Motion Sensor : fl_lib/Mechanical/Mechanical Sensors/Ideal Rotational Motion Sensor  reference=foundation.enum.MeasurementReference.difference  acceleration_port=false  velocity_port=true  position_port=true  wrap_angle=simscape.enum.onoff.off  offset=0 rad
  PS-Simulink Converter3 : nesl_utility/PS-Simulink Converter  PhysicalDomain=network_engine_domain  SubClassName=ps_output  LeftPortType=input  RightPortType=output  PseudoPeriodic=off  Frequencies=[]  VectorFormat=1-D array  Unit=rpm  AffineConversion=off
  Zero-Order Hold : ZeroOrderHold  SampleTime=0.01
  F : PMIOPort  Side=Right
  B : PMIOPort  Port=2  Side=Left
  S1 : Outport  VectorParamsAs1DForOutWhenUnconnected=off
  wires:
  PS-Simulink Converter3/1 -> Zero-Order Hold/1
  Zero-Order Hold/1 -> S1/1
  connections:
  Ideal Rotational Motion Sensor/RConn2 -- PS-Simulink Converter3/LConn1
  F/RConn1 -- Ideal Rotational Motion Sensor/RConn1
  B/RConn1 -- Ideal Rotational Motion Sensor/LConn1

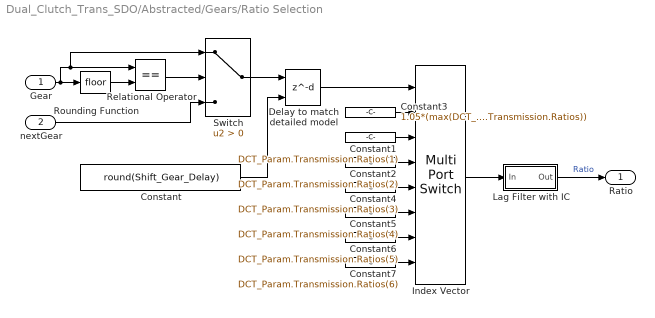
== system Dual_Clutch_Trans_SDO/Abstracted/Gears/Ratio Selection ==
  Gear : Inport
  nextGear : Inport  Port=2
  Constant : Constant  Value=round(Shift_Gear_Delay)  OutDataTypeStr=int8
  Constant1 : Constant  Value=DCT_Param.Transmission.Ratios(1)
  Constant2 : Constant  Value=DCT_Param.Transmission.Ratios(2)
  Constant3 : Constant  Value=1.05*(max(DCT_Param.Transmission.Ratios))
  Constant4 : Constant  Value=DCT_Param.Transmission.Ratios(3)
  Constant5 : Constant  Value=DCT_Param.Transmission.Ratios(4)
  Constant6 : Constant  Value=DCT_Param.Transmission.Ratios(5)
  Constant7 : Constant  Value=DCT_Param.Transmission.Ratios(6)
  Delay to match detailed model : Delay  DelayLengthSource=Input port  DelayLength=round(Shift_Gear_Delay)  InitialCondition=1  SampleTime=0.01
      settings: InputPortMap=u0,p1
  Index Vector : MultiPortSwitch  DataPortOrder=Zero-based contiguous  Inputs=7  zeroidx=on  SaturateOnIntegerOverflow=off  InputSameDT=off
  Lag Filter with IC : Subsystem  mask(First-order lag supporting vector signals){b=Ratio_Time_Const, x_initial=DCT_Param.Transmission.Ratios(1)}
      mask prompts: b "Filter time constant"; x_initial "Initial output"
      mask help: Models a lag of the form 1/(b*s+1) where s is the Laplace operator.
  Relational Operator : RelationalOperator  Operator===  OutDataTypeStr=boolean  InputSameDT=off
  Rounding Function : Rounding
  Switch : Switch  Criteria=u2 > Threshold  SaturateOnIntegerOverflow=off  InputSameDT=off
  Ratio : Outport  VectorParamsAs1DForOutWhenUnconnected=off
  wires:
  Delay to match detailed model/1 -> Index Vector/1
  nextGear/1 -> Switch/3
  Switch/1 -> Delay to match detailed model/1
  Relational Operator/1 -> Switch/2
  Rounding Function/1 -> Relational Operator/2
  Lag Filter with IC/1(Out) -> Ratio/1  "Ratio"
  Gear/1 -> Switch/1, Relational Operator/1, Rounding Function/1
  Constant3/1 -> Index Vector/2
  Constant1/1 -> Index Vector/3
  Constant2/1 -> Index Vector/4
  Constant4/1 -> Index Vector/5
  Constant5/1 -> Index Vector/6
  Constant6/1 -> Index Vector/7
  Constant7/1 -> Index Vector/8
  Index Vector/1 -> Lag Filter with IC/1(In)
  Constant/1 -> Delay to match detailed model/2

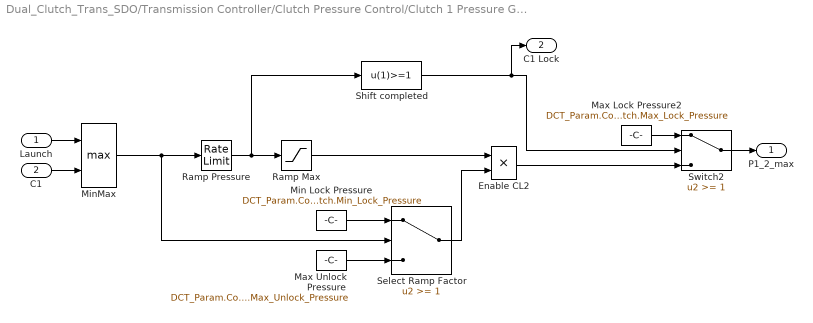
== system Dual_Clutch_Trans_SDO/Transmission Controller/Clutch Pressure Control/Clutch 1 Pressure Gears 2 through max ==
  Launch : Inport
  C1 : Inport  Port=2
  Enable CL2 : Product  InputSameDT=on  SaturateOnIntegerOverflow=on  OutDataTypeStr=Inherit: Same as first input
  Max Lock Pressure2 : Constant  Value=DCT_Param.Control.Clutch.Max_Lock_Pressure  SampleTime=0.01
  Max Unlock Pressure : Constant  Value=DCT_Param.Control.Clutch.Max_Unlock_Pressure  SampleTime=0.01
  Min Lock Pressure : Constant  Value=DCT_Param.Control.Clutch.Min_Lock_Pressure  SampleTime=0.01
  MinMax : MinMax  Function=max  Inputs=2
  Ramp Pressure : RateLimiter  RisingSlewLimit=1/0.5  FallingSlewLimit=-1/0.5  SampleTimeMode=inherited
  Ramp Max : Saturate  UpperLimit=1/0.5  LowerLimit=0
  Select Ramp Factor : Switch  Threshold=1  SaturateOnIntegerOverflow=off  InputSameDT=off
  Shift completed : Fcn  Expr=u(1)>=1  SampleTime=0.01
  Switch2 : Switch  Threshold=1  SaturateOnIntegerOverflow=off  InputSameDT=off
  P1_2_max : Outport  VectorParamsAs1DForOutWhenUnconnected=off
  C1 Lock : Outport  Port=2  VectorParamsAs1DForOutWhenUnconnected=off
  wires:
  Launch/1 -> MinMax/1
  C1/1 -> MinMax/2
  Shift completed/1 -> Switch2/2, C1 Lock/1
  Ramp Max/1 -> Enable CL2/1
  Ramp Pressure/1 -> Ramp Max/1, Shift completed/1
  Max Unlock Pressure/1 -> Select Ramp Factor/3
  Min Lock Pressure/1 -> Select Ramp Factor/1
  Select Ramp Factor/1 -> Enable CL2/2
  Enable CL2/1 -> Switch2/3
  Max Lock Pressure2/1 -> Switch2/1
  MinMax/1 -> Select Ramp Factor/2, Ramp Pressure/1
  Switch2/1 -> P1_2_max/1

== system Dual_Clutch_Trans_SDO/Transmission Controller/Clutch Pressure Control/Clutch 1 Pressure Launch ==
  Pedal : Inport
  Launch : Inport  Port=2
  P1_2_max : Inport  Port=3
  1/(0.18s+1) to allow for engine lag : DiscreteTransferFcn  Numerator=0.054  Denominator=[1 -0.946]  SampleTime=0.01
  Inverse clutch model : Subsystem  mask(Inverse clutch model){r_eff=0.13, N=4, A=0.001, mu=0.3}
      mask prompts: r_eff "Effective torque radius (m)"; N "Number of friction surfaces"; A "Engagement piston area (m^2)"; mu "Kinetic friction coefficient"
      mask help: Converts the demanded input torque into the required clutch pressure.
  Switch5 : Switch  Threshold=1  SaturateOnIntegerOverflow=off  InputSameDT=off
  Tmax : Gain  Gain=92e3/(2*pi*5500/60)  SaturateOnIntegerOverflow=on  OutDataTypeStr=Inherit: Same as input  ParamDataTypeStr=Inherit: Same as input
  P1_dem : Outport  VectorParamsAs1DForOutWhenUnconnected=off
  wires:
  Launch/1 -> Switch5/2
  Inverse clutch model/1(P) -> Switch5/1  "P_Launch"
  Pedal/1 -> Tmax/1
  1/(0.18s+1) to allow for engine lag/1 -> Inverse clutch model/1(Trq)
  Tmax/1 -> 1/(0.18s+1) to allow for engine lag/1
  Switch5/1 -> P1_dem/1
  P1_2_max/1 -> Switch5/3

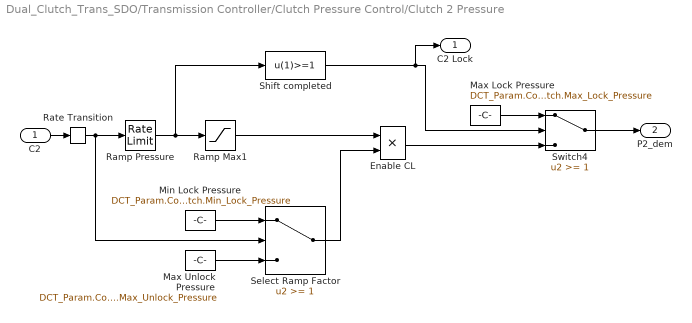
== system Dual_Clutch_Trans_SDO/Transmission Controller/Clutch Pressure Control/Clutch 2 Pressure ==
  C2 : Inport
  Enable CL : Product  InputSameDT=on  SaturateOnIntegerOverflow=on  OutDataTypeStr=Inherit: Same as first input
  Max Lock Pressure : Constant  Value=DCT_Param.Control.Clutch.Max_Lock_Pressure  SampleTime=0.01
  Max Unlock Pressure : Constant  Value=DCT_Param.Control.Clutch.Max_Unlock_Pressure  SampleTime=0.01
  Min Lock Pressure : Constant  Value=DCT_Param.Control.Clutch.Min_Lock_Pressure  SampleTime=0.01
  Ramp Pressure : RateLimiter  RisingSlewLimit=1/0.5  FallingSlewLimit=-1/0.5  SampleTimeMode=inherited
  Ramp Max1 : Saturate  UpperLimit=1/0.5  LowerLimit=0
  Rate Transition : RateTransition  OutPortSampleTime=0.01
  Select Ramp Factor : Switch  Threshold=1  SaturateOnIntegerOverflow=off  InputSameDT=off
  Shift completed : Fcn  Expr=u(1)>=1  SampleTime=0.01
  Switch4 : Switch  Threshold=1  SaturateOnIntegerOverflow=off  InputSameDT=off
  C2 Lock : Outport  VectorParamsAs1DForOutWhenUnconnected=off
  P2_dem : Outport  Port=2  VectorParamsAs1DForOutWhenUnconnected=off
  wires:
  Rate Transition/1 -> Select Ramp Factor/2, Ramp Pressure/1
  Shift completed/1 -> Switch4/2, C2 Lock/1
  Enable CL/1 -> Switch4/3
  Max Lock Pressure/1 -> Switch4/1
  Select Ramp Factor/1 -> Enable CL/2
  Min Lock Pressure/1 -> Select Ramp Factor/1
  Max Unlock Pressure/1 -> Select Ramp Factor/3
  Ramp Pressure/1 -> Shift completed/1, Ramp Max1/1
  Ramp Max1/1 -> Enable CL/1
  Switch4/1 -> P2_dem/1
  C2/1 -> Rate Transition/1

== system Dual_Clutch_Trans_SDO/Transmission Controller/Driver/Open Loop Tests ==
  Cmd_Br : Inport
  Cmd_Pd : Inport  Port=2
  Compare To Constant : simulink/Logic and Bit Operations/Compare To Constant  relop===  const=6  OutDataTypeStr=uint8
  Demux : Demux  Outputs=2
  Open Loop Brake : Switch  Criteria=u2 > Threshold  SaturateOnIntegerOverflow=off  InputSameDT=off
  Open Loop Throttle : Switch  Criteria=u2 > Threshold  SampleTime=0.01  SaturateOnIntegerOverflow=off  InputSameDT=off
  Select Cycle : Constant  Value=Drive_Cycle_Num  SampleTime=0.01
  Step : Step  Time=[30 30]  Before=[0 1]  After=[-550 0]  SampleTime=0
  Brake : Outport  VectorParamsAs1DForOutWhenUnconnected=off
  Pedal : Outport  Port=2  VectorParamsAs1DForOutWhenUnconnected=off
  wires:
  Compare To Constant/1 -> Open Loop Brake/2, Open Loop Throttle/2
  Step/1 -> Demux/1
  Select Cycle/1 -> Compare To Constant/1
  Open Loop Brake/1 -> Brake/1  "Brake"
  Cmd_Br/1 -> Open Loop Brake/3
  Open Loop Throttle/1 -> Pedal/1  "Acc"
  Cmd_Pd/1 -> Open Loop Throttle/3
  Demux/2 -> Open Loop Throttle/1
  Demux/1 -> Open Loop Brake/1

== system Dual_Clutch_Trans_SDO/Transmission Controller/Gear shift demands/Actuator 1 demand ==
  P : Inport
  nG : Inport  Port=2
  Disengage : Constant  Value=-1
  Engage : Constant
  Pulse sign : Switch  Threshold=0.5  SaturateOnIntegerOverflow=off
  Signed pulse : Product  InputSameDT=on  SaturateOnIntegerOverflow=on  OutDataTypeStr=Inherit: Same as first input
  Pulse : Outport  VectorParamsAs1DForOutWhenUnconnected=off
  wires:
  nG/1 -> Pulse sign/2
  P/1 -> Signed pulse/1
  Signed pulse/1 -> Pulse/1
  Pulse sign/1 -> Signed pulse/2
  Engage/1 -> Pulse sign/1
  Disengage/1 -> Pulse sign/3

== system Dual_Clutch_Trans_SDO/Transmission Controller/Gear shift demands/Actuator 2 demand ==
  P : Inport
  nG : Inport  Port=2
  Disengage : Constant  Value=-1
  Engage : Constant
  Pulse sign : Switch  Threshold=0.5  SaturateOnIntegerOverflow=off
  Signed pulse : Product  InputSameDT=on  SaturateOnIntegerOverflow=on  OutDataTypeStr=Inherit: Same as first input
  Pulse : Outport  VectorParamsAs1DForOutWhenUnconnected=off
  wires:
  Disengage/1 -> Pulse sign/3
  Engage/1 -> Pulse sign/1
  Pulse sign/1 -> Signed pulse/2
  Signed pulse/1 -> Pulse/1
  P/1 -> Signed pulse/1
  nG/1 -> Pulse sign/2

== system Dual_Clutch_Trans_SDO/Transmission Controller/Gear shift demands/Actuator 3 demand ==
  P : Inport
  nG : Inport  Port=2
  Disengage : Constant  Value=-1
  Engage : Constant
  Pulse sign : Switch  Threshold=0.5  SaturateOnIntegerOverflow=off
  Signed pulse : Product  InputSameDT=on  SaturateOnIntegerOverflow=on  OutDataTypeStr=Inherit: Same as first input
  Pulse : Outport  VectorParamsAs1DForOutWhenUnconnected=off
  wires:
  Disengage/1 -> Pulse sign/3
  Engage/1 -> Pulse sign/1
  Pulse sign/1 -> Signed pulse/2
  Signed pulse/1 -> Pulse/1
  P/1 -> Signed pulse/1
  nG/1 -> Pulse sign/2

== system Dual_Clutch_Trans_SDO/Transmission Controller/Gear shift demands/Actuator 4 demand ==
  P : Inport
  nG : Inport  Port=2
  Disengage : Constant  Value=-1
  Engage : Constant
  Pulse sign : Switch  Threshold=0.5  SaturateOnIntegerOverflow=off
  Signed pulse : Product  InputSameDT=on  SaturateOnIntegerOverflow=on  OutDataTypeStr=Inherit: Same as first input
  Pulse : Outport  VectorParamsAs1DForOutWhenUnconnected=off
  wires:
  nG/1 -> Pulse sign/2
  P/1 -> Signed pulse/1
  Signed pulse/1 -> Pulse/1
  Pulse sign/1 -> Signed pulse/2
  Engage/1 -> Pulse sign/1
  Disengage/1 -> Pulse sign/3

== system Dual_Clutch_Trans_SDO/Transmission Controller/Gear shift demands/Actuator 5 demand ==
  P : Inport
  nG : Inport  Port=2
  Disengage : Constant  Value=-1
  Engage : Constant
  Pulse sign : Switch  Threshold=0.5  SaturateOnIntegerOverflow=off
  Signed pulse : Product  InputSameDT=on  SaturateOnIntegerOverflow=on  OutDataTypeStr=Inherit: Same as first input
  Pulse : Outport  VectorParamsAs1DForOutWhenUnconnected=off
  wires:
  nG/1 -> Pulse sign/2
  P/1 -> Signed pulse/1
  Signed pulse/1 -> Pulse/1
  Pulse sign/1 -> Signed pulse/2
  Engage/1 -> Pulse sign/1
  Disengage/1 -> Pulse sign/3

== system Dual_Clutch_Trans_SDO/Transmission Controller/Gear shift demands/Actuator 6 demand ==
  P : Inport
  nG : Inport  Port=2
  Disengage : Constant  Value=-1
  Engage : Constant
  Pulse sign : Switch  Threshold=0.5  SaturateOnIntegerOverflow=off
  Signed pulse : Product  InputSameDT=on  SaturateOnIntegerOverflow=on  OutDataTypeStr=Inherit: Same as first input
  Pulse : Outport  VectorParamsAs1DForOutWhenUnconnected=off
  wires:
  Disengage/1 -> Pulse sign/3
  Engage/1 -> Pulse sign/1
  Pulse sign/1 -> Signed pulse/2
  Signed pulse/1 -> Pulse/1
  P/1 -> Signed pulse/1
  nG/1 -> Pulse sign/2

== system Dual_Clutch_Trans_SDO/Transmission Controller/Gear shift demands/Create pulse if next gear number changes and CL1 is not engaged ==
  ~E : Inport
  nG : Inport  Port=2
  0.5s delay : Delay  DelayLength=DCT_Param.Dog_Clutches.Pulse_Length  SampleTime=0.01
  Abs : Abs
  Create a 1/2s pulse if not engaged and the next gear number changes : Product  InputSameDT=on  SaturateOnIntegerOverflow=on  OutDataTypeStr=Inherit: Same as first input
  Rate Transition : RateTransition  OutPortSampleTime=0.01
  Rate Transition2 : RateTransition  OutPortSampleTime=0.01
  Sum2 : Sum  Inputs=|+-  InputSameDT=on  SaturateOnIntegerOverflow=on  OutDataTypeStr=Inherit: Same as first input
  "[0,1]" : Saturate  UpperLimit=1  LowerLimit=0
  Pulse : Outport  VectorParamsAs1DForOutWhenUnconnected=off
  wires:
  Rate Transition2/1 -> 0.5s delay/1, Sum2/2
  Rate Transition/1 -> Create a 1/2s pulse if not engaged and the next gear number changes/1
  ~E/1 -> Create a 1/2s pulse if not engaged and the next gear number changes/2
  Create a 1/2s pulse if not engaged and the next gear number changes/1 -> Pulse/1
  "[0,1]"/1 -> Rate Transition/1
  Abs/1 -> "[0,1]"/1
  Sum2/1 -> Abs/1
  0.5s delay/1 -> Sum2/1
  nG/1 -> Rate Transition2/1
